simulink model "ur5_ctc"  (R2026b)
settings: Solver=ode45  StopTime=Tend  MaxStep=1e-3  RelTol=1e-5
undefined symbols (not defined in the file): KdC, KiC, KpC, NB, NBc, q0, sigmaQ, sigmaQd, tauMax
libraries: robotmaniplib x2
settings Model: Creator=har  LastModifiedBy=har

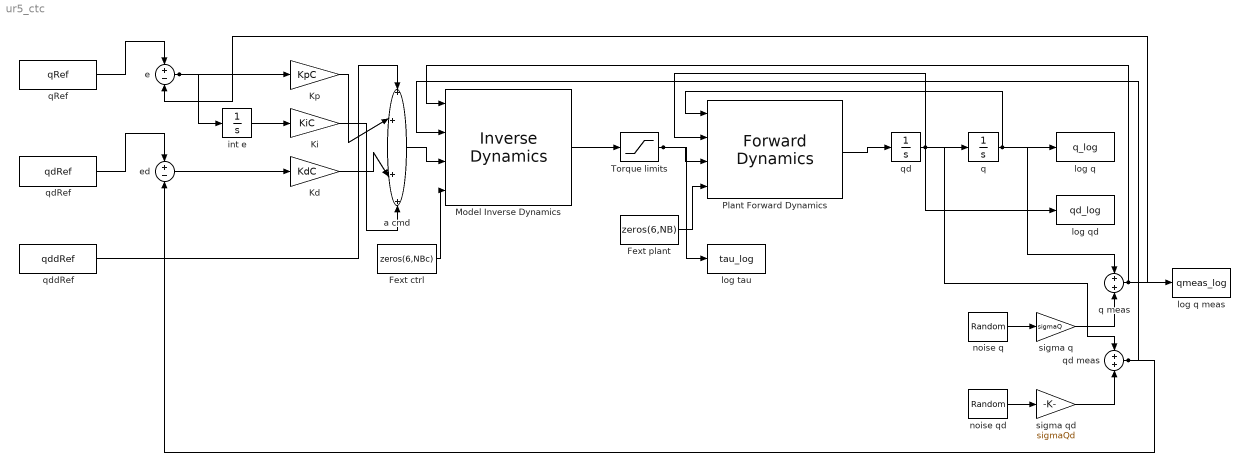
== system ur5_ctc ==
  Fext ctrl : Constant  Value=zeros(6,NBc)
  Fext plant : Constant  Value=zeros(6,NB)
  Kd : Gain  Gain=KdC
  Ki : Gain  Gain=KiC
  Kp : Gain  Gain=KpC
  Model Inverse Dynamics : robotmaniplib/Inverse Dynamics  RigidBodyTree=robotCtrl  SimulateUsing=Code generation
  Plant Forward Dynamics : robotmaniplib/Forward Dynamics  RigidBodyTree=robotPlant  SimulateUsing=Code generation
  Torque limits : Saturate  UpperLimit=tauMax  LowerLimit=-tauMax
  a cmd : Sum  Inputs=++++
  e : Sum  Inputs=+-
  ed : Sum  Inputs=+-
  int e : Integrator  InitialCondition=zeros(6,1)
  log q : ToWorkspace  VariableName=q_log  SaveFormat=Timeseries  SampleTime=-1
  log q meas : ToWorkspace  VariableName=qmeas_log  SaveFormat=Timeseries  SampleTime=-1
  log qd : ToWorkspace  VariableName=qd_log  SaveFormat=Timeseries  SampleTime=-1
  log tau : ToWorkspace  VariableName=tau_log  SaveFormat=Timeseries  SampleTime=-1
  noise q : RandomNumber  Mean=zeros(6,1)  Variance=ones(6,1)  Seed=[11 12 13 14 15 16]  SampleTime=1e-3
  noise qd : RandomNumber  Mean=zeros(6,1)  Variance=ones(6,1)  Seed=[21 22 23 24 25 26]  SampleTime=1e-3
  q : Integrator  InitialCondition=q0
  q meas : Sum
  qRef : FromWorkspace  VariableName=qRef  OutputAfterFinalValue=Holding final value
  qd : Integrator  InitialCondition=zeros(6,1)
  qd meas : Sum
  qdRef : FromWorkspace  VariableName=qdRef  OutputAfterFinalValue=Holding final value
  qddRef : FromWorkspace  VariableName=qddRef  OutputAfterFinalValue=Holding final value
  sigma q : Gain  Gain=sigmaQ
  sigma qd : Gain  Gain=sigmaQd
  wires:
  q/1 -> q meas/1, Plant Forward Dynamics/1, log q/1
  noise q/1 -> sigma q/1
  sigma q/1 -> q meas/2
  qd/1 -> qd meas/1, Plant Forward Dynamics/2, q/1, log qd/1
  noise qd/1 -> sigma qd/1
  sigma qd/1 -> qd meas/2
  qRef/1 -> e/1
  q meas/1 -> e/2, Model Inverse Dynamics/1, log q meas/1
  qdRef/1 -> ed/1
  qd meas/1 -> ed/2, Model Inverse Dynamics/2
  e/1 -> int e/1, Kp/1
  int e/1 -> Ki/1
  ed/1 -> Kd/1
  qddRef/1 -> a cmd/1
  Kp/1 -> a cmd/2
  Kd/1 -> a cmd/3
  Ki/1 -> a cmd/4
  a cmd/1 -> Model Inverse Dynamics/3
  Fext ctrl/1 -> Model Inverse Dynamics/4
  Model Inverse Dynamics/1 -> Torque limits/1
  Torque limits/1 -> Plant Forward Dynamics/3, log tau/1
  Fext plant/1 -> Plant Forward Dynamics/4
  Plant Forward Dynamics/1 -> qd/1
